simulink model "LabA_LinearizedBotVsSimulator"  (R2026b)
settings: Solver=ode14x  StopTime=5  FixedStep=0.001  RelTol=1e-2  EnableMultiTasking=on
values from neighbouring files (symbols this model uses):
  A = [0, 1, 0, 0 ... (first row only)    [LabA_equations.m]    (also in LabA_parameters.mat = [0 0 0 0 1 0.0716665297455 0 0.0185556406229 0 0.01784481592; LabB_ObserverAndControllerOverSimulator_Continuous_Parameters.m = 1.0e+03 * [; matlab.mat = [0 0 0 0 1 -435.034344762 0 1903.43949265 0 -6.0990753006 0 )
  Bd = [0,           0 ... (first row only)    [LabA_equations.m]    (also in LabB_ObserverOverSimulator_Discrete_Parameters.m = [)
  Cf = eye(4)    [LabA_equations.m]
  D_bd = zeros(4, 2)    [LabA_equations.m]
  Kd_val = (alpha2 - a2) / b1    [LabA_equations.m]
  Ki_val = (alpha0 - a0) / b1    [LabA_equations.m]
  Kp_val = (alpha1 - a1) / b1    [LabA_equations.m]
libraries: slpidlib x2, cstblocks_lti x1
settings Model: Creator=The MathWorks Inc.  LastModifiedBy=holyk
settings DataIOCC: LimitDataPoints=on  ReturnWorkspaceOutputs=off  SaveFormat=Array  SignalLoggingName=logsOut
settings OptimizationCC: EfficientMapNaN2IntZero=off  MemsetInitFltsAndDblsToZero=off
settings DebuggingCC: ArithmeticOperatorsInVariantConditions=warning  FcnCallInpInsideContextMsg=warning  MergeDetectMultiDrivingBlocksExec=none  SFExecutionAtInitializationDiag=none  SFNoUnconditionalDefaultTransitionDiag=warning  SFUnexpectedBacktrackingDiag=warning  SignalResolutionControl=TryResolveAllWithWarning  StateNameClashWarn=warning  UnderspecifiedInitializationDetection=Classic
settings HardwareCC: ProdHWDeviceType=Intel->x86-64 (Linux 64)  ProdLongLongMode=on  TargetEndianess=LittleEndian  TargetHWDeviceType=Intel->x86-64  TargetIntDivRoundTo=Zero
settings ModelReferenceCC: PropagateSignalLabelsOutOfModel=off
settings SFSimCC: CustomCodeUndefinedFunction=UseInterfaceOnly  SimUseLocalCustomCode=off
settings RTWCC: Description=Simulink Desktop Real-Time  RTWCompilerOptimization=on  RTWUseLocalCustomCode=off  SystemTargetFile=sldrt.tlc  TemplateMakefile=sldrt.tmf
settings CodeAppCC: StateflowObjectComments=on
settings SimulinkDesktopRealTimeCC: ParMdlRefBuildCompliant=on  RealTimeExecution=kernel  TargetLangStandard=C89/C90 (ANSI)  TargetLibSuffix=_sldrt.a  TargetPreCompLibLocation=C:\Program Files\MATLAB\R2026b\toolbox\sldrt\lib\win64
settings ConfigComp: CovExternalEMLEnable=off  CovSFcnEnable=off  CovSaveCumulativeToWorkspaceVar=on  CovSaveSingleToWorkspaceVar=on

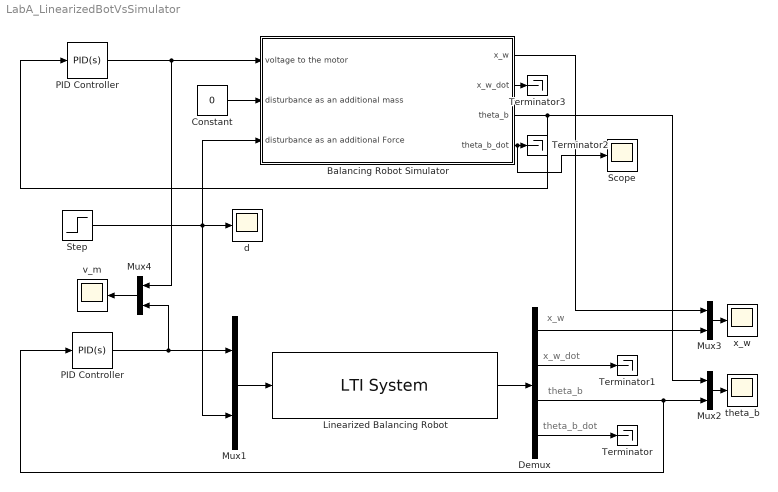
== system LabA_LinearizedBotVsSimulator ==
  note: x_w_dot
  note: x_w
  note: theta_b
  note: theta_b_dot
  Balancing Robot Simulator : Subsystem  mask(Balancing Robot Simulator Parameters){g=9.8, m_b=0.381, l_b=0.112, I_b=0.00616, m_w=0.036, l_w=0.021, I_w=0.00000746, R_m=4.4, L_m=0, b_m=0, b_f=0, K_e=0.444, K_t=0.470, X_0=0, x_w=2.0295, Theta=2.5696e-12, circle_x=0, circle_y=0, scale=2, v_m_limit=9, Theta_0=0*pi/180, x_w_0=0, sigma2_angle=0}
      mask prompts: g "gravitational acceleration"; m_b "mass of the body [kg]"; l_b "length of the body [m]"; I_b "moment of inertia of the body [kg m^2]"; m_w "mass of the wheels [kg]"; l_w "radius of the wheels [m]"; I_w "moment of inertia of the wheels [kg m^2]"; R_m "electrical resistance of the motor [Ohm]"; L_m "electrical inductance of the motor [Henry]"; b_m "viscuous coefficient of the motor"; b_f "wheels - ground friction coefficient"; K_e "back EMF constant of the motor"; K_t "torque constant of the motor"; circle_x "Circl_x"; circle_y "Circl_y"; v_m_limit "saturation limits for the motor voltage"; Theta_0 "initial angle of the body"; x_w_0 "initial position of the wheels"; sigma2_angle "variance of the angle measurement noise"
      mask init:
      | hBlk=get_param(gcb,'Handle');
      | 
      | X_0=[Theta_0 0 x_w_0 0];
      | %%% calculate the circle
      | 
      | r=l_w ;
      | x=-r:r/10:r;
      | circle_y=r*[sqrt(1-x.^2/r^2), -sqrt(1-x.^2/r^2) ]+r;
      | circle_x=[x,x([length(x):-1:1])];
      mask DialogControl PhysicalParametersTab Prompt: Physical parameters
      mask DialogControl InitialConditionsTab Prompt: Initial conditions
      mask DialogControl MeasurementsSystemParametersTab Prompt: Measurement system parameters
      mask Display:
      | color('black');
      | plot([0.0,0.0,1 ,1,0 ],[1,0,0,1,1])
      | port_label('input',		1,  'motor voltage')
      | port_label('input',		2,  'additional mass')
      | port_label('input',		3,  'additional force')
      | port_label('output',	1,	'x_w')
      | port_label('output',	2,	'x_w_dot')
      | port_label('output',	3,	'theta_b')
      | port_label('output',	4,	'theta_b_dot')
      | 
      | x_b = x_w + l_b * sin(Theta);
      | y_b = l_w + l_b * cos(Theta);
      | 
      | Y_OFF = 0.1;
      | X_OFF = 0.5;
      | 
      | plot([0.05,0.95],[Y_OFF,Y_OFF])
      | plot([0.5,0.5],[Y_OFF/2,Y_OFF])
      | 
      | color('r');
      | plot(	(circle_x+x_w)*scale +X_OFF,	...
      | 		(circle_y)*scale+Y_OFF			);
      | 
      | plot(	[x_w x_b] * scale + X_OFF,	...
      | 		[l_w y_b] * scale + Y_OFF	);
      | 
      | color('r');
      | text(0.5, 0.5,																	...
      | 	['theta_b = ' num2str(Theta*180/pi,3) char(10) 'x_w = ' num2str(x_w,3)],		...
      | 	'HorizontalAlignment',	'center',											...
      |     'VerticalAlignment',	'bottom'											);
  Constant : Constant  Value=0
  Demux : Demux
  Linearized Balancing Robot : cstblocks_lti/LTI System  sys=ss(A,Bd,Cf,D_bd)  IC=[0 0 0*pi/180 0]  PadeOrder=0
  Mux{1..4} (4 alike) : Mux  Inputs=2
  PID Controller : slpidlib/PID Controller  Controller=PID  Form=Parallel  TimeDomain=Continuous-time  UseExternalTs=off  SampleTime=-1  IntegratorMethod=Forward Euler  FilterMethod=Forward Euler  ControllerParametersSource=internal  P=-Kp_val  I=-Ki_val  UseKiTs=off  D=-Kd_val  UseExternalDerivativeSource=off  N=100000  UseFilter=on  TunerSelectOption=Transfer Function Based (PID Tuner App)  InitialConditionSource=internal  InitialConditionForIntegrator=0  InitialConditionForFilter=0  DifferentiatorICPrevScaledInput=0  ExternalReset=none  TrackingMode=off  Kt=1  LimitOutput=on  SatLimitsSource=internal  UpperSaturationLimit=9  LowerSaturationLimit=-9  LinearizeAsGain=on  AntiWindupMode=clamping  Kb=1  LimitIntegrator=off  UpperIntegratorSaturationLimit=inf  LowerIntegratorSaturationLimit=-inf  POutMin=[]  POutMax=[]  IOutMin=[]  IOutMax=[]  DOutMin=[]  DOutMax=[]  NOutMin=[]  NOutMax=[]  SumOutMin=[]  SumOutMax=[]  SaturationOutMin=[]  SaturationOutMax=[]  PParamMin=[]  PParamMax=[]  IParamMin=[]  IParamMax=[]  DParamMin=[]  DParamMax=[]  NParamMin=[]  NParamMax=[]  KbParamMin=[]  KbParamMax=[]  KtParamMin=[]  KtParamMax=[]  KbOutMin=[]  KbOutMax=[]  KtOutMin=[]  KtOutMax=[]  IntegratorOutMin=[]  IntegratorOutMax=[]  FilterOutMin=[]  FilterOutMax=[]  SumI1OutMin=[]  SumI1OutMax=[]  SumI2OutMin=[]  SumI2OutMax=[]  SumI3OutMin=[]  SumI3OutMax=[]  SumI4OutMin=[]  SumI4OutMax=[]  SumDOutMin=[]  SumDOutMax=[]  DifferentiatorOutMin=[]  DifferentiatorOutMax=[]  FilterDiffOutCoefMin=[]  FilterDiffOutCoefMax=[]  ReciprocalOutMin=[]  ReciprocalOutMax=[]  SumDenOutMin=[]  SumDenOutMax=[]  SumNumOutMin=[]  SumNumOutMax=[]  DivideOutMin=[]  DivideOutMax=[]  UdiffTsProdOutMin=[]  UdiffTsProdOutMax=[]  NTsProdOutMin=[]  NTsProdOutMax=[]  UintegralTsProdOutMin=[]  UintegralTsProdOutMax=[]  UngainTsProdOutMin=[]  UngainTsProdOutMax=[]  ClampingZeroOutDataTypeStr=Inherit: Inherit via back propagation  ClampingZeroOutMin=[]  ClampingZeroOutMax=[]  FilterDenConstantOutDataTypeStr=Inherit: Inherit via back propagation  FilterDenConstantOutMin=[]  FilterDenConstantOutMax=[]  PCopyOutDataTypeStr=Inherit: Inherit via back propagation  PCopyOutMin=[]  PCopyOutMax=[]  NCopyOutDataTypeStr=Inherit: Inherit via back propagation  NCopyOutMin=[]  NCopyOutMax=[]  IntegratorContinuousStateAttributes=''  IntegratorStateMustResolveToSignalObject=off  IntegratorRTWStateStorageClass=Auto  FilterContinuousStateAttributes=''  FilterStateMustResolveToSignalObject=off  FilterRTWStateStorageClass=Auto  ParallelPVariant=InternalParameters  IdealPVariant=Disabled  IVariant=InternalParameters  DVariant=InternalParameters  IntegratorVariant=Continuous  SatVariant=Enabled  AWVariant=ContClampingParallel  PCopyVariant=Disabled  TRVariant=Disabled  FdbkBlocksVariant=Forward  IdealPFdbkVariant=Disabled  SatFdbkVariant=Disabled  DerivativeFilterVariant=ContFilter  NVariant=InternalParameters  NCopyVariant=Disabled  FilterICVariant=InternalICsFilter  IntegratorICVariant=InternalICs  ExternalResetVariant=Disabled  TRSumVariant=Passthrough  SumFdbkVariant=Disabled  SumVariant=Sum_PID  TsampFilterVariant=InternalTs  TsampNgainVariant=Passthrough  TsampIntegralVariant=Disabled_SignalSpec  ExternalSaturationOutDataTypeStr=Inherit: Same as second input  DerivativeSourceVariant=ErrorSignal  PreIntVariant=InternalPreInt
  "PID Controller " : slpidlib/PID Controller  Controller=PID  Form=Parallel  TimeDomain=Continuous-time  UseExternalTs=off  SampleTime=-1  IntegratorMethod=Forward Euler  FilterMethod=Forward Euler  ControllerParametersSource=internal  P=-Kp_val  I=-Ki_val  UseKiTs=off  D=-Kd_val  UseExternalDerivativeSource=off  N=100000  UseFilter=on  TunerSelectOption=Transfer Function Based (PID Tuner App)  InitialConditionSource=internal  InitialConditionForIntegrator=0  InitialConditionForFilter=0  DifferentiatorICPrevScaledInput=0  ExternalReset=none  TrackingMode=off  Kt=1  LimitOutput=off  SatLimitsSource=internal  UpperSaturationLimit=inf  LowerSaturationLimit=-inf  LinearizeAsGain=on  AntiWindupMode=none  Kb=1  LimitIntegrator=off  UpperIntegratorSaturationLimit=inf  LowerIntegratorSaturationLimit=-inf  POutMin=[]  POutMax=[]  IOutMin=[]  IOutMax=[]  DOutMin=[]  DOutMax=[]  NOutMin=[]  NOutMax=[]  SumOutMin=[]  SumOutMax=[]  SaturationOutMin=[]  SaturationOutMax=[]  PParamMin=[]  PParamMax=[]  IParamMin=[]  IParamMax=[]  DParamMin=[]  DParamMax=[]  NParamMin=[]  NParamMax=[]  KbParamMin=[]  KbParamMax=[]  KtParamMin=[]  KtParamMax=[]  KbOutMin=[]  KbOutMax=[]  KtOutMin=[]  KtOutMax=[]  IntegratorOutMin=[]  IntegratorOutMax=[]  FilterOutMin=[]  FilterOutMax=[]  SumI1OutMin=[]  SumI1OutMax=[]  SumI2OutMin=[]  SumI2OutMax=[]  SumI3OutMin=[]  SumI3OutMax=[]  SumI4OutMin=[]  SumI4OutMax=[]  SumDOutMin=[]  SumDOutMax=[]  DifferentiatorOutMin=[]  DifferentiatorOutMax=[]  FilterDiffOutCoefMin=[]  FilterDiffOutCoefMax=[]  ReciprocalOutMin=[]  ReciprocalOutMax=[]  SumDenOutMin=[]  SumDenOutMax=[]  SumNumOutMin=[]  SumNumOutMax=[]  DivideOutMin=[]  DivideOutMax=[]  UdiffTsProdOutMin=[]  UdiffTsProdOutMax=[]  NTsProdOutMin=[]  NTsProdOutMax=[]  UintegralTsProdOutMin=[]  UintegralTsProdOutMax=[]  UngainTsProdOutMin=[]  UngainTsProdOutMax=[]  ClampingZeroOutDataTypeStr=Inherit: Inherit via back propagation  ClampingZeroOutMin=[]  ClampingZeroOutMax=[]  FilterDenConstantOutDataTypeStr=Inherit: Inherit via back propagation  FilterDenConstantOutMin=[]  FilterDenConstantOutMax=[]  PCopyOutDataTypeStr=Inherit: Inherit via back propagation  PCopyOutMin=[]  PCopyOutMax=[]  NCopyOutDataTypeStr=Inherit: Inherit via back propagation  NCopyOutMin=[]  NCopyOutMax=[]  IntegratorContinuousStateAttributes=''  IntegratorStateMustResolveToSignalObject=off  IntegratorRTWStateStorageClass=Auto  FilterContinuousStateAttributes=''  FilterStateMustResolveToSignalObject=off  FilterRTWStateStorageClass=Auto  ParallelPVariant=InternalParameters  IdealPVariant=Disabled  IVariant=InternalParameters  DVariant=InternalParameters  IntegratorVariant=Continuous  SatVariant=Disabled  AWVariant=Passthrough  PCopyVariant=Disabled  TRVariant=Disabled  FdbkBlocksVariant=Forward  IdealPFdbkVariant=Disabled  SatFdbkVariant=Disabled  DerivativeFilterVariant=ContFilter  NVariant=InternalParameters  NCopyVariant=Disabled  FilterICVariant=InternalICsFilter  IntegratorICVariant=InternalICs  ExternalResetVariant=Disabled  TRSumVariant=Passthrough  SumFdbkVariant=Disabled  SumVariant=Sum_PID  TsampFilterVariant=InternalTs  TsampNgainVariant=Passthrough  TsampIntegralVariant=Disabled_SignalSpec  ExternalSaturationOutDataTypeStr=Inherit: Same as second input  DerivativeSourceVariant=ErrorSignal  PreIntVariant=InternalPreInt
  Scope : Scope
      settings: ActiveDisplayYMinimum=-1.207030254992872  ActiveDisplayYMaximum=9.72305873896284
  Step : Step  Time=0.1  InitialValue=0.827  FinalValue=0  SampleTime=0
  Terminator{,1..3} (4 alike) : Terminator
  d : Scope
      settings: ActiveDisplayYMinimum=-0.10349999999999997  ActiveDisplayYMaximum=0.9315  DataLoggingVariableName=d
  theta_b : Scope
      settings: ActiveDisplayYMinimum=-0.19643575851539385  ActiveDisplayYMaximum=1.7679218266385452  DataLoggingVariableName=theta_b
  v_m : Scope
      settings: ActiveDisplayYMinimum=-1.1142043570027567  ActiveDisplayYMaximum=10.027839213024812  DataLoggingVariableName=v_m
  x_w : Scope
      settings: ActiveDisplayYMinimum=-0.30649138534664461  ActiveDisplayYMaximum=2.758422468119802  DataLoggingVariableName=x_w
  wires:
  PID Controller/1 -> Mux4/1, Balancing Robot Simulator/1(voltage to the motor)
  Mux1/1 -> Linearized Balancing Robot/1
  Linearized Balancing Robot/1 -> Demux/1
  Step/1 -> Mux1/2, Balancing Robot Simulator/3(disturbance as an additional Force), d/1
  Balancing Robot Simulator/3(theta_b) -> Mux2/1, PID Controller/1
  Balancing Robot Simulator/1(x_w) -> Mux3/1
  Mux3/1 -> x_w/1
  Mux2/1 -> theta_b/1
  Demux/1 -> Mux3/2
  Demux/3 -> Mux2/2, "PID Controller "/1
  "PID Controller "/1 -> Mux4/2, Mux1/1
  Mux4/1 -> v_m/1
  Demux/2 -> Terminator1/1
  Demux/4 -> Terminator/1
  Balancing Robot Simulator/4("theta_b_dot ") -> Scope/1, Terminator2/1
  Balancing Robot Simulator/2(x_w_dot) -> Terminator3/1
  Constant/1 -> Balancing Robot Simulator/2("disturbance as an additional mass ")

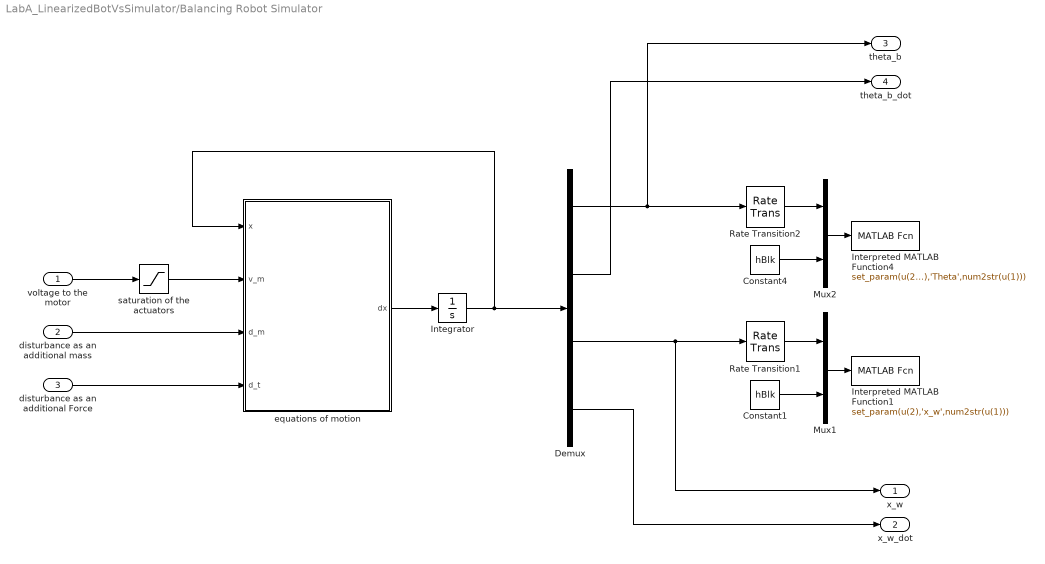
== system LabA_LinearizedBotVsSimulator/Balancing Robot Simulator ==
  voltage to the motor : Inport
  "disturbance as an additional mass " : Inport  Port=2
  disturbance as an additional Force : Inport  Port=3
  Constant1 : Constant  Value=hBlk
  Constant4 : Constant  Value=hBlk
  Demux : Demux
  Integrator : Integrator  InitialCondition=X_0
  Interpreted MATLAB Function1 : MATLABFcn  MATLABFcn=set_param(u(2),'x_w',num2str(u(1)))  OutputDimensions=0  SampleTime=0.1
  Interpreted MATLAB Function4 : MATLABFcn  MATLABFcn=set_param(u(2),'Theta',num2str(u(1)))  OutputDimensions=0
  Mux1 : Mux  Inputs=2
  Mux2 : Mux  Inputs=2
  Rate Transition1 : RateTransition  OutPortSampleTime=0.1
  Rate Transition2 : RateTransition  OutPortSampleTime=0.1
  equations of motion : MATLAB Function  TreatAsAtomicUnit=on
  saturation of the actuators : Saturate  UpperLimit=v_m_limit  LowerLimit=-v_m_limit
  x_w : Outport
  x_w_dot : Outport  Port=2
  theta_b : Outport  Port=3
  "theta_b_dot " : Outport  Port=4
  wires:
  Integrator/1 -> equations of motion/1(x), Demux/1
  Constant4/1 -> Mux2/2
  Mux2/1 -> Interpreted MATLAB Function4/1
  Rate Transition2/1 -> Mux2/1
  equations of motion/1(dx) -> Integrator/1
  voltage to the motor/1 -> saturation of the actuators/1
  Constant1/1 -> Mux1/2
  Mux1/1 -> Interpreted MATLAB Function1/1
  Rate Transition1/1 -> Mux1/1
  Demux/3 -> x_w/1, Rate Transition1/1
  saturation of the actuators/1 -> equations of motion/2(v_m)
  "disturbance as an additional mass "/1 -> equations of motion/3(d_m)
  disturbance as an additional Force/1 -> equations of motion/4(d_t)
  Demux/1 -> theta_b/1, Rate Transition2/1
  Demux/2 -> "theta_b_dot "/1
  Demux/4 -> x_w_dot/1

== matlab function LabA_LinearizedBotVsSimulator/Balancing Robot Simulator/equations of motion ==
  data: x input; dx output; v_m input; d_m input; d_t input; g parameter; b_f parameter; m_b parameter; l_b parameter; I_b parameter; m_w parameter; l_w parameter; I_w parameter; R_m parameter; L_m parameter; b_m parameter; K_e parameter; K_t parameter
function dx = EquationsOfMotion(x,		...
								v_m,	...
								d_m,	... % additional mass on the body
								d_t,	... % Fource that acted on the body
								g,		...
								b_f,	...
								m_b,	...
								l_b,	...
								I_b,	...
								m_w,	...
								l_w,	...
								I_w,	...
								R_m,	...
								L_m,	...
								b_m,	...
								K_e,	...
								K_t		) %#ok<*INUSL>

% initialization of the state
dx = zeros(4,1);

% TODO: the motor electrical inductance and the motor viscous coefficients
% are neglected

% for readability -- state of the system
theta		= x(1);
theta_dot	= x(2);
x_b			= x(3);
x_b_dot		= x(4);

% add the mass disturbance: notice that we need to modify also the
% moment of inertia
m_t_b = m_b + d_m;
I_t_b = I_b * m_t_b / m_b;

% equations of motion (obfuscated)
dx(1)=theta_dot;
dx(2)=((b_f + (K_e*K_t)/R_m)*(theta_dot - x_b_dot/l_w) + (K_t*v_m)/R_m - d_t*l_b*1*cos(theta) - g*l_b*m_t_b*sin(theta) + (l_b*m_t_b*cos(theta)*(d_t*l_w + (b_f + (K_e*K_t)/R_m)*(theta_dot - x_b_dot/l_w) + (K_t*v_m)/R_m + l_b*l_w*m_t_b*theta_dot^2*sin(theta)))/(l_w*m_t_b + l_w*m_w + I_w/l_w))/((m_t_b*l_b^2 + I_t_b)*((l_b^2*l_w*m_t_b^2*cos(theta)^2)/((m_t_b*l_b^2 + I_t_b)*(l_w*m_t_b + l_w*m_w + I_w/l_w)) - 1));
dx(3)=x_b_dot;
dx(4)= -(d_t*l_w + (b_f + (K_e*K_t)/R_m)*(theta_dot - x_b_dot/l_w) + (K_t*v_m)/R_m + l_b*l_w*m_t_b*theta_dot^2*sin(theta) + (l_b*l_w*m_t_b*cos(theta)*((b_f + (K_e*K_t)/R_m)*(theta_dot - x_b_dot/l_w) + (K_t*v_m)/R_m - d_t*l_b*1*cos(theta) - g*l_b*m_t_b*sin(theta)))/(m_t_b*l_b^2 + I_t_b))/(((l_b^2*l_w*m_t_b^2*cos(theta)^2)/((m_t_b*l_b^2 + I_t_b)*(l_w*m_t_b + l_w*m_w + I_w/l_w)) - 1)*(l_w*m_t_b + l_w*m_w + I_w/l_w));

% if the robot falls
if( (x(1) > pi/2) || (x(1) < -pi/2) )
	%
	dx(1) = 0;
	dx(2) = 0;
	dx(3) = 0;
	dx(4) = 0;
	%
end;%


% g   = 9.8;
% b_f = 0;
% m_t_b = 0.381;
% l_b = 0.112;
% I_t_b = 0.00616;
% m_w = 0.036;
% l_w = 0.021;
% I_w = 0.00000746;
% R_m = 4.4;
% L_m = 0 ;
% b_m = 0;
% K_e = 0.444;
% K_t = 0.470;
